simulink model "MotorFaultDetector"  (R2026a)
settings: Solver=FixedStepDiscrete  StopTime=7.9999  FixedStep=1/12000
settings Model: Creator=Tejashri  LastModifiedBy=Tejashri

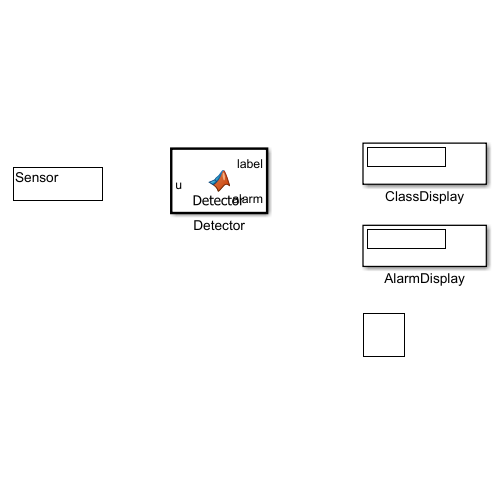
[thumbnail: Simulink's stored preview of the top-level diagram]
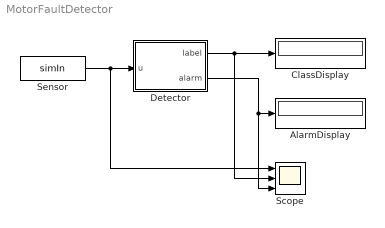
== system MotorFaultDetector ==
  AlarmDisplay : Display
  ClassDisplay : Display
  Detector : MATLAB Function  TreatAsAtomicUnit=on
  Scope : Scope  NumInputPorts=3
  Sensor : FromWorkspace  VariableName=simIn  SampleTime=1/12000  OutputAfterFinalValue=Holding final value
  wires:
  Sensor/1 -> Scope/1, Detector/1(u)
  Detector/1(label) -> Scope/2, ClassDisplay/1
  Detector/2(alarm) -> Scope/3, AlarmDisplay/1

== matlab function MotorFaultDetector/Detector ==
  data: u input; label output; alarm output
function [label, alarm] = Detector(u)
[label, alarm] = motorDetector(u);
